simulink model "Controller"  (R2018b)
settings: configuration reference "control_config" (kept outside this file)
values from neighbouring files (symbols this model uses):
  CONTROL_EXPORT = Simulink.Parameter(CONTROL_EXPORT_VALUE)    [controller_model_init.m]
  CONTROL_PARAM = Simulink.Parameter(CONTROL_PARAM_VALUE)    [controller_model_init.m]
undefined symbols (not defined in the file or in its folder): actuator_cmd, ControlMode, DiscIntNeverNeededParam, timestamp
libraries: FMT_Model_Lib x4, simulink x3
settings Model: Creator=jc  LastModifiedBy=zouji
settings ConfigSetRef: SourceLocation=Base Workspace

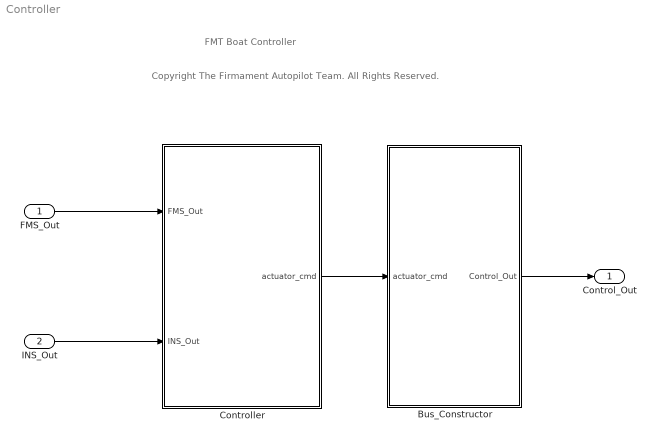
== system Controller ==
  note: FMT Boat Controller
  note: Copyright The Firmament Autopilot Team. All Rights Reserved.
  FMS_Out : Inport  OutDataTypeStr=Bus: FMS_Out_Bus
  INS_Out : Inport  Port=2  OutDataTypeStr=Bus: INS_Out_Bus
  Bus_Constructor : Subsystem
  Controller : Subsystem
  Control_Out : Outport  OutDataTypeStr=Bus: Control_Out_Bus
  wires:
  Bus_Constructor/1(Control_Out) -> Control_Out/1
  INS_Out/1 -> Controller/2(INS_Out)
  FMS_Out/1 -> Controller/1(FMS_Out)
  Controller/1(actuator_cmd) -> Bus_Constructor/1(actuator_cmd)

== system Controller/Bus_Constructor ==
  actuator_cmd : Inport
  Bus Assignment : BusAssignment  AssignedSignals=actuator_cmd,timestamp
  Constant : Constant  Value=0  OutDataTypeStr=Bus: Control_Out_Bus
  timestamp : Subsystem  mask{sample_time=CONTROL_EXPORT.period}
      mask prompts: sample_time "sample time (ms)"
  Control_Out : Outport
  wires:
  actuator_cmd/1 -> Bus Assignment/2
  Constant/1 -> Bus Assignment/1
  Bus Assignment/1 -> Control_Out/1
  timestamp/1(timestamp_ms) -> Bus Assignment/3

== system Controller/Controller ==
  FMS_Out : Inport
  INS_Out : Inport  Port=2
  Control_Allocation : Subsystem  Variant=on
      settings: GeneratePreprocessorConditionals=on
  Heading_Controller : Subsystem
  Speed_Controller : Subsystem
  actuator_cmd : Outport
  wires:
  FMS_Out/1 -> Speed_Controller/1(FMS_Out), Heading_Controller/2(FMS_Out), Control_Allocation/3(FMS_Out)
  INS_Out/1 -> Heading_Controller/1(INS_Out), Speed_Controller/2(INS_Out)
  Control_Allocation/1(actuator_cmd) -> actuator_cmd/1
  Speed_Controller/1(throttle_cmd) -> Control_Allocation/1(throttle_cmd)  "throttle_cmd"
  Heading_Controller/1(steering_cmd) -> Control_Allocation/2(steering_cmd)  "steering_cmd"

== system Controller/Bus_Constructor/timestamp ==
  Constant : Constant  Value=sample_time
  Data Type Conversion : DataTypeConversion  OutDataTypeStr=uint32
  Discrete-Time Integrator : DiscreteIntegrator  IntegratorMethod=Accumulation: Forward Euler  SampleTime=-1  ICPrevOutput=DiscIntNeverNeededParam  ICPrevScaledInput=DiscIntNeverNeededParam
  timestamp_ms : Outport
  wires:
  Discrete-Time Integrator/1 -> Data Type Conversion/1
  Constant/1 -> Discrete-Time Integrator/1
  Data Type Conversion/1 -> timestamp_ms/1

== system Controller/Controller/Control_Allocation ==
  note: 1) Add Subsystem or Model blocks as valid variant choices.
      | 2) You cannot connect blocks at this level. At simulation, connectivity is automatically
      | determined, based on the active variant and port name matching.
  throttle_cmd : Inport
  steering_cmd : Inport  Port=2
  FMS_Out : Inport  Port=3
  Boat_1 : Subsystem  TreatAsAtomicUnit=on  VariantControl=AIRFRAME==1
      mask Display: image('D:\ws\FMT\FMT-Model\figures\boat_1.png');
  Boat_2 : Subsystem  TreatAsAtomicUnit=on  VariantControl=AIRFRAME==2
      mask Display: image('D:\ws\FMT\FMT-Model\figures\boat_1.png');
  actuator_cmd : Outport

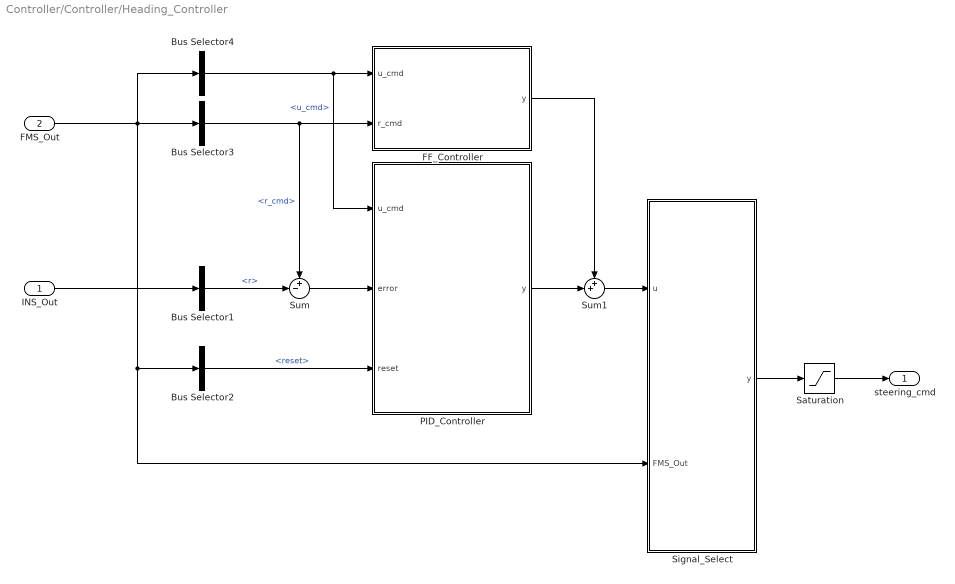
== system Controller/Controller/Heading_Controller ==
  INS_Out : Inport
  FMS_Out : Inport  Port=2
  Bus Selector1 : BusSelector  OutputSignals=r
  Bus Selector2 : BusSelector  OutputSignals=reset
  Bus Selector3 : BusSelector  OutputSignals=r_cmd
  Bus Selector4 : BusSelector  OutputSignals=u_cmd
  FF_Controller : Subsystem
  PID_Controller : Subsystem
  Saturation : Saturate  UpperLimit=1  LowerLimit=-1
  Signal_Select : Subsystem
  Sum : Sum  Inputs=+-|
  Sum1 : Sum  Inputs=++|
  steering_cmd : Outport
  wires:
  Bus Selector2/1 -> PID_Controller/3(reset)  "<reset>"
  Sum/1 -> PID_Controller/2(error)
  FMS_Out/1 -> Bus Selector4/1, Signal_Select/2(FMS_Out), Bus Selector2/1, Bus Selector3/1
  Bus Selector3/1 -> Sum/1, FF_Controller/2(r_cmd)  "<r_cmd>"
  INS_Out/1 -> Bus Selector1/1
  Bus Selector1/1 -> Sum/2  "<r>"
  PID_Controller/1(y) -> Sum1/2
  Signal_Select/1(y) -> Saturation/1
  Saturation/1 -> steering_cmd/1
  Sum1/1 -> Signal_Select/1(u)
  Bus Selector4/1 -> FF_Controller/1(u_cmd), PID_Controller/1(u_cmd)  "<u_cmd>"
  FF_Controller/1(y) -> Sum1/1

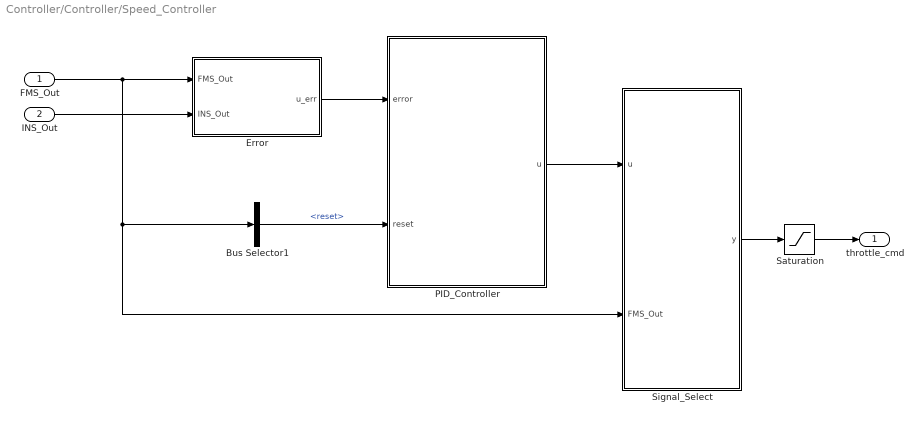
== system Controller/Controller/Speed_Controller ==
  FMS_Out : Inport
  INS_Out : Inport  Port=2
  Bus Selector1 : BusSelector  OutputSignals=reset
  Error : Subsystem
  PID_Controller : Subsystem
  Saturation : Saturate  UpperLimit=1  LowerLimit=-1
  Signal_Select : Subsystem
  throttle_cmd : Outport
  wires:
  Bus Selector1/1 -> PID_Controller/2(reset)  "<reset>"
  FMS_Out/1 -> Signal_Select/2(FMS_Out), Bus Selector1/1, Error/1(FMS_Out)
  Error/1(u_err) -> PID_Controller/1(error)
  PID_Controller/1(u) -> Signal_Select/1(u)
  INS_Out/1 -> Error/2(INS_Out)
  Signal_Select/1(y) -> Saturation/1
  Saturation/1 -> throttle_cmd/1

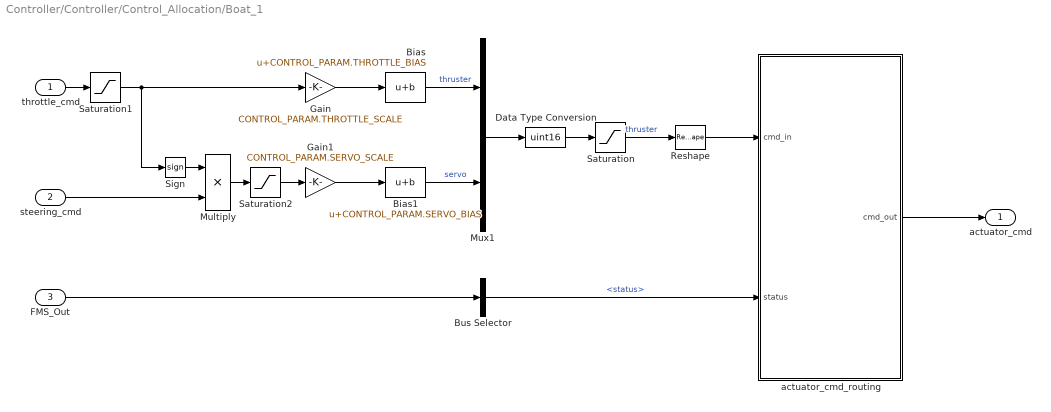
== system Controller/Controller/Control_Allocation/Boat_1 ==
  throttle_cmd : Inport
  steering_cmd : Inport  Port=2
  FMS_Out : Inport  Port=3
  Bias : Bias  Bias=CONTROL_PARAM.THROTTLE_BIAS
  Bias1 : Bias  Bias=CONTROL_PARAM.SERVO_BIAS
  Bus Selector : BusSelector  OutputSignals=status
  Data Type Conversion : DataTypeConversion  OutDataTypeStr=uint16
  Gain : Gain  Gain=CONTROL_PARAM.THROTTLE_SCALE  OutDataTypeStr=single
  Gain1 : Gain  Gain=CONTROL_PARAM.SERVO_SCALE  OutDataTypeStr=single
  Multiply : Product
  Mux1 : Mux  Inputs=2
  Reshape : Reshape  OutputDimensionality=Column vector (2-D)
  Saturation : Saturate  UpperLimit=2000  LowerLimit=1000
  Saturation1 : Saturate  UpperLimit=CONTROL_PARAM.THROTTLE_MAX  LowerLimit=CONTROL_PARAM.THROTTLE_MIN
  Saturation2 : Saturate  UpperLimit=CONTROL_PARAM.SERVO_MAX  LowerLimit=CONTROL_PARAM.SERVO_MIN
  Sign : Signum
  actuator_cmd_routing : Subsystem
  actuator_cmd : Outport
  wires:
  Bias1/1 -> Mux1/2  "servo"
  Gain1/1 -> Bias1/1
  Gain/1 -> Bias/1
  steering_cmd/1 -> Multiply/2
  Bias/1 -> Mux1/1  "thruster"
  Bus Selector/1 -> actuator_cmd_routing/2(status)  "<status>"
  Reshape/1 -> actuator_cmd_routing/1(cmd_in)
  FMS_Out/1 -> Bus Selector/1
  Mux1/1 -> Data Type Conversion/1
  actuator_cmd_routing/1(cmd_out) -> actuator_cmd/1
  Saturation/1 -> Reshape/1  "thruster"
  Data Type Conversion/1 -> Saturation/1
  throttle_cmd/1 -> Saturation1/1
  Saturation2/1 -> Gain1/1
  Multiply/1 -> Saturation2/1
  Sign/1 -> Multiply/1
  Saturation1/1 -> Sign/1, Gain/1

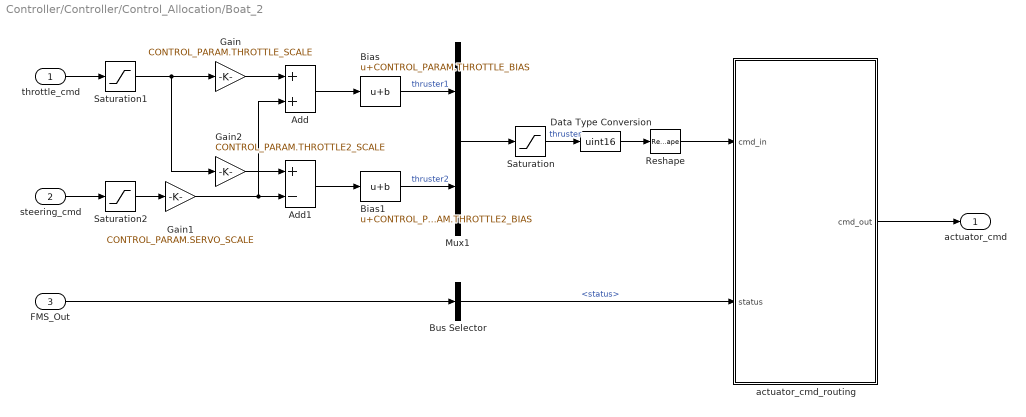
== system Controller/Controller/Control_Allocation/Boat_2 ==
  throttle_cmd : Inport
  steering_cmd : Inport  Port=2
  FMS_Out : Inport  Port=3
  Add : Sum
  Add1 : Sum  Inputs=+-
  Bias : Bias  Bias=CONTROL_PARAM.THROTTLE_BIAS
  Bias1 : Bias  Bias=CONTROL_PARAM.THROTTLE2_BIAS
  Bus Selector : BusSelector  OutputSignals=status
  Data Type Conversion : DataTypeConversion  OutDataTypeStr=uint16
  Gain : Gain  Gain=CONTROL_PARAM.THROTTLE_SCALE  OutDataTypeStr=single
  Gain1 : Gain  Gain=CONTROL_PARAM.SERVO_SCALE  OutDataTypeStr=single
  Gain2 : Gain  Gain=CONTROL_PARAM.THROTTLE2_SCALE  OutDataTypeStr=single
  Mux1 : Mux  Inputs=2
  Reshape : Reshape  OutputDimensionality=Column vector (2-D)
  Saturation : Saturate  UpperLimit=2000  LowerLimit=1000
  Saturation1 : Saturate  UpperLimit=CONTROL_PARAM.THROTTLE_MAX  LowerLimit=CONTROL_PARAM.THROTTLE_MIN
  Saturation2 : Saturate  UpperLimit=CONTROL_PARAM.SERVO_MAX  LowerLimit=CONTROL_PARAM.SERVO_MIN
  actuator_cmd_routing : Subsystem
  actuator_cmd : Outport
  wires:
  Bias1/1 -> Mux1/2  "thruster2"
  throttle_cmd/1 -> Saturation1/1
  Bias/1 -> Mux1/1  "thruster1"
  Bus Selector/1 -> actuator_cmd_routing/2(status)  "<status>"
  Reshape/1 -> actuator_cmd_routing/1(cmd_in)
  FMS_Out/1 -> Bus Selector/1
  actuator_cmd_routing/1(cmd_out) -> actuator_cmd/1
  Saturation/1 -> Data Type Conversion/1  "thruster"
  Mux1/1 -> Saturation/1
  steering_cmd/1 -> Saturation2/1
  Saturation1/1 -> Gain2/1, Gain/1
  Data Type Conversion/1 -> Reshape/1
  Add1/1 -> Bias1/1
  Add/1 -> Bias/1
  Gain/1 -> Add/1
  Gain1/1 -> Add/2, Add1/2
  Saturation2/1 -> Gain1/1
  Gain2/1 -> Add1/1

== system Controller/Controller/Heading_Controller/FF_Controller ==
  u_cmd : Inport
  r_cmd : Inport  Port=2
  BW_FF : Gain  Gain=CONTROL_PARAM.BW_PSI_RATE_FF
  FW_FF : Gain  Gain=CONTROL_PARAM.FW_PSI_RATE_FF
  Saturation : Saturate  UpperLimit=1  LowerLimit=-1
  Switch : Switch
  y : Outport
  wires:
  r_cmd/1 -> BW_FF/1, FW_FF/1
  FW_FF/1 -> Switch/1
  BW_FF/1 -> Switch/3
  Switch/1 -> Saturation/1
  u_cmd/1 -> Switch/2
  Saturation/1 -> y/1

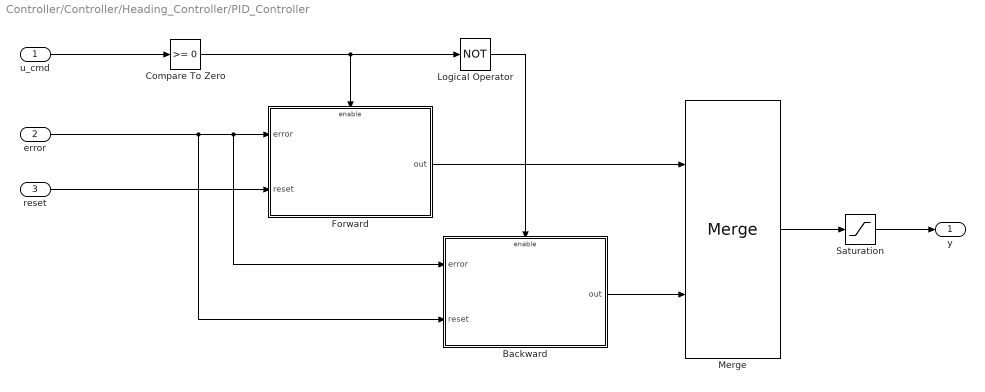
== system Controller/Controller/Heading_Controller/PID_Controller ==
  u_cmd : Inport
  error : Inport  Port=2
  reset : Inport  Port=3
  Backward : Subsystem
  Compare To Zero : simulink/Logic and Bit Operations/Compare To Zero  relop=>=  OutDataTypeStr=boolean
  Forward : Subsystem
  Logical Operator : Logic  Operator=NOT  AllPortsSameDT=off  OutDataTypeStr=boolean
  Merge : Merge
  Saturation : Saturate  UpperLimit=1  LowerLimit=-1
  y : Outport
  wires:
  Saturation/1 -> y/1
  error/1 -> Backward/2(reset), Backward/1(error), Forward/1(error)
  reset/1 -> Forward/2(reset)
  u_cmd/1 -> Compare To Zero/1
  Compare To Zero/1 -> Logical Operator/1, Forward/Enable
  Logical Operator/1 -> Backward/Enable
  Backward/1(out) -> Merge/2
  Forward/1(out) -> Merge/1
  Merge/1 -> Saturation/1

== system Controller/Controller/Heading_Controller/Signal_Select ==
  u : Inport
  FMS_Out : Inport  Port=2
  Bus Selector : BusSelector  OutputSignals=ctrl_mode
  Bus Selector1 : BusSelector  OutputSignals=r_cmd
  Position : simulink/Logic and Bit Operations/Compare To Constant  relop=>=  const=uint8(ControlMode.Stabilize)  OutDataTypeStr=boolean
  Switch : Switch  Criteria=u2 > Threshold
  y : Outport
  wires:
  FMS_Out/1 -> Bus Selector1/1, Bus Selector/1
  Bus Selector/1 -> Position/1  "<ctrl_mode>"
  Position/1 -> Switch/2
  Switch/1 -> y/1
  u/1 -> Switch/1
  Bus Selector1/1 -> Switch/3  "<r_cmd>"

== system Controller/Controller/Speed_Controller/Error ==
  FMS_Out : Inport
  INS_Out : Inport  Port=2
  Bus Selector2 : BusSelector  OutputSignals=u_cmd
  Bus_Select : Subsystem
  Sum : Sum  Inputs=|+-
  u_err : Outport
  wires:
  FMS_Out/1 -> Bus Selector2/1
  INS_Out/1 -> Bus_Select/1(INS_Out)
  Bus_Select/1(u_est_C_mPs) -> Sum/2  "u_est"
  Bus Selector2/1 -> Sum/1  "<u_cmd>"
  Sum/1 -> u_err/1  "u_err"

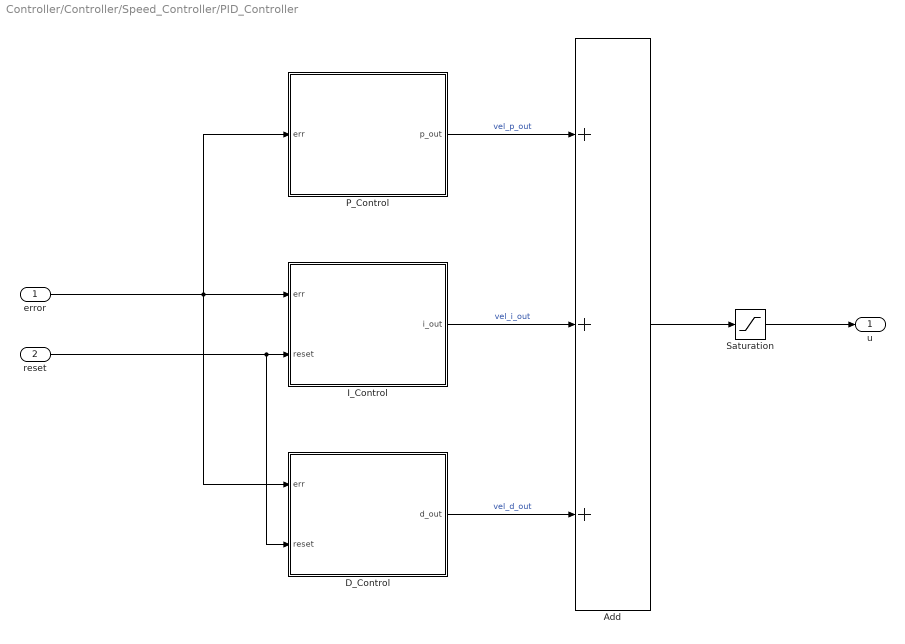
== system Controller/Controller/Speed_Controller/PID_Controller ==
  error : Inport
  reset : Inport  Port=2
  Add : Sum  Inputs=+++
  D_Control : Subsystem  mask{kd=CONTROL_PARAM.VEL_D, max_d=CONTROL_PARAM.VEL_D_MAX, min_d=CONTROL_PARAM.VEL_D_MIN}
  I_Control : Subsystem  mask{ki=CONTROL_PARAM.VEL_I, max_i=CONTROL_PARAM.VEL_I_MAX, min_i=CONTROL_PARAM.VEL_I_MIN}
  P_Control : Subsystem  mask{kp=CONTROL_PARAM.VEL_P}
  Saturation : Saturate  UpperLimit=1  LowerLimit=-1
  u : Outport
  wires:
  error/1 -> P_Control/1(err), I_Control/1(err), D_Control/1(err)
  P_Control/1(p_out) -> Add/1  "vel_p_out"
  I_Control/1(i_out) -> Add/2  "vel_i_out"
  D_Control/1(d_out) -> Add/3  "vel_d_out"
  reset/1 -> I_Control/2(reset), D_Control/2(reset)
  Add/1 -> Saturation/1
  Saturation/1 -> u/1

== system Controller/Controller/Speed_Controller/Signal_Select ==
  u : Inport
  FMS_Out : Inport  Port=2
  Bus Selector : BusSelector  OutputSignals=ctrl_mode
  Bus Selector1 : BusSelector  OutputSignals=u_cmd
  Position : simulink/Logic and Bit Operations/Compare To Constant  relop=>=  const=uint8(ControlMode.POSCTL)  OutDataTypeStr=boolean
  Switch : Switch  Criteria=u2 > Threshold
  y : Outport
  wires:
  FMS_Out/1 -> Bus Selector1/1, Bus Selector/1
  Bus Selector/1 -> Position/1  "<ctrl_mode>"
  Position/1 -> Switch/2
  Switch/1 -> y/1
  u/1 -> Switch/1
  Bus Selector1/1 -> Switch/3  "<u_cmd>"

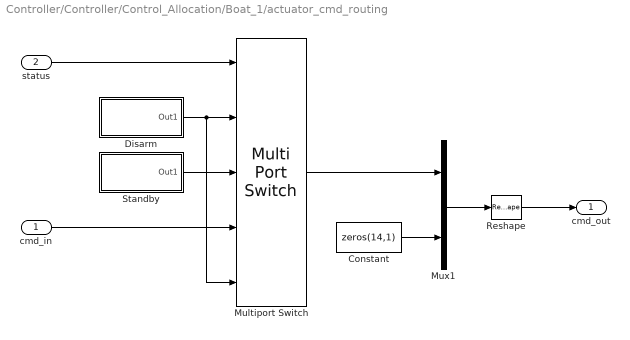
== system Controller/Controller/Control_Allocation/Boat_1/actuator_cmd_routing ==
  cmd_in : Inport
  status : Inport  Port=2
  Constant : Constant  Value=zeros(14,1)  VectorParams1D=off  OutDataTypeStr=uint16
  Disarm : Subsystem
  Multiport Switch : MultiPortSwitch  DataPortForDefault=Additional data port  DiagnosticForDefault=None
  Mux1 : Mux  Inputs=2
  Reshape : Reshape  OutputDimensionality=Customize  OutputDimensions=[16,1]
  Standby : Subsystem
  cmd_out : Outport
  wires:
  Reshape/1 -> cmd_out/1
  Constant/1 -> Mux1/2
  Mux1/1 -> Reshape/1
  status/1 -> Multiport Switch/1
  Multiport Switch/1 -> Mux1/1
  cmd_in/1 -> Multiport Switch/4
  Disarm/1(Out1) -> Multiport Switch/5, Multiport Switch/2
  Standby/1(Out1) -> Multiport Switch/3

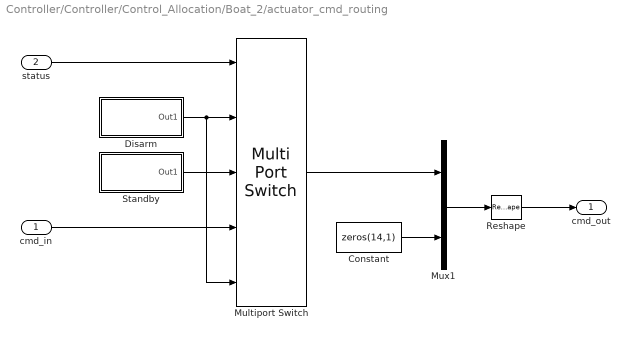
== system Controller/Controller/Control_Allocation/Boat_2/actuator_cmd_routing ==
  cmd_in : Inport
  status : Inport  Port=2
  Constant : Constant  Value=zeros(14,1)  VectorParams1D=off  OutDataTypeStr=uint16
  Disarm : Subsystem
  Multiport Switch : MultiPortSwitch  DataPortForDefault=Additional data port  DiagnosticForDefault=None
  Mux1 : Mux  Inputs=2
  Reshape : Reshape  OutputDimensionality=Customize  OutputDimensions=[16,1]
  Standby : Subsystem
  cmd_out : Outport
  wires:
  Reshape/1 -> cmd_out/1
  Constant/1 -> Mux1/2
  Mux1/1 -> Reshape/1
  status/1 -> Multiport Switch/1
  Multiport Switch/1 -> Mux1/1
  cmd_in/1 -> Multiport Switch/4
  Disarm/1(Out1) -> Multiport Switch/5, Multiport Switch/2
  Standby/1(Out1) -> Multiport Switch/3

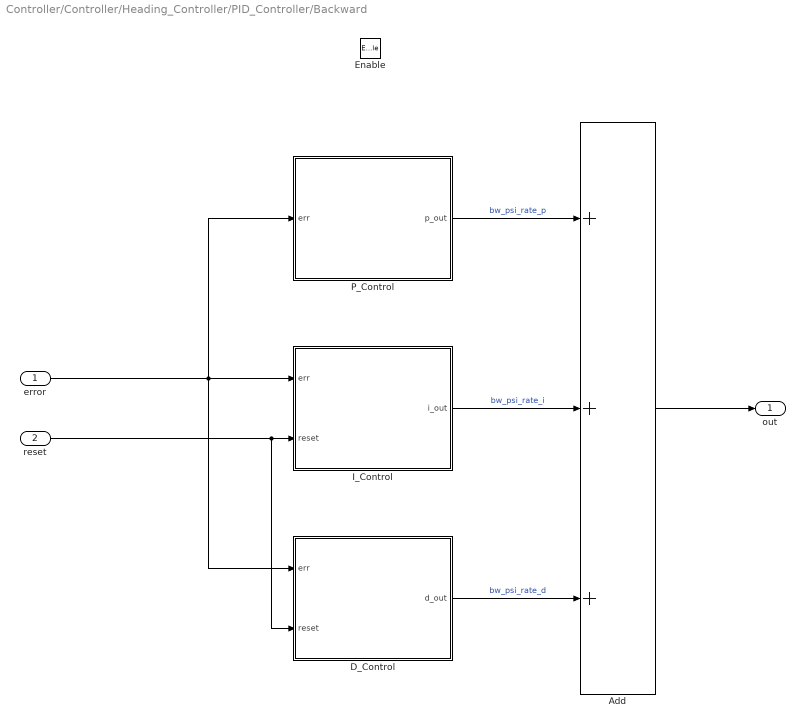
== system Controller/Controller/Heading_Controller/PID_Controller/Backward ==
  error : Inport
  reset : Inport  Port=2
  Enable : EnablePort  StatesWhenEnabling=reset
  Add : Sum  Inputs=+++
  D_Control : Subsystem  mask{kd=CONTROL_PARAM.BW_PSI_RATE_D, max_d=0.2, min_d=-0.2}
  I_Control : Subsystem  mask{ki=CONTROL_PARAM.BW_PSI_RATE_I, max_i=0.2, min_i=-0.2}
  P_Control : Subsystem  mask{kp=CONTROL_PARAM.BW_PSI_RATE_P}
  out : Outport
  wires:
  I_Control/1(i_out) -> Add/2  "bw_psi_rate_i"
  D_Control/1(d_out) -> Add/3  "bw_psi_rate_d"
  Add/1 -> out/1
  reset/1 -> D_Control/2(reset), I_Control/2(reset)
  P_Control/1(p_out) -> Add/1  "bw_psi_rate_p"
  error/1 -> D_Control/1(err), I_Control/1(err), P_Control/1(err)

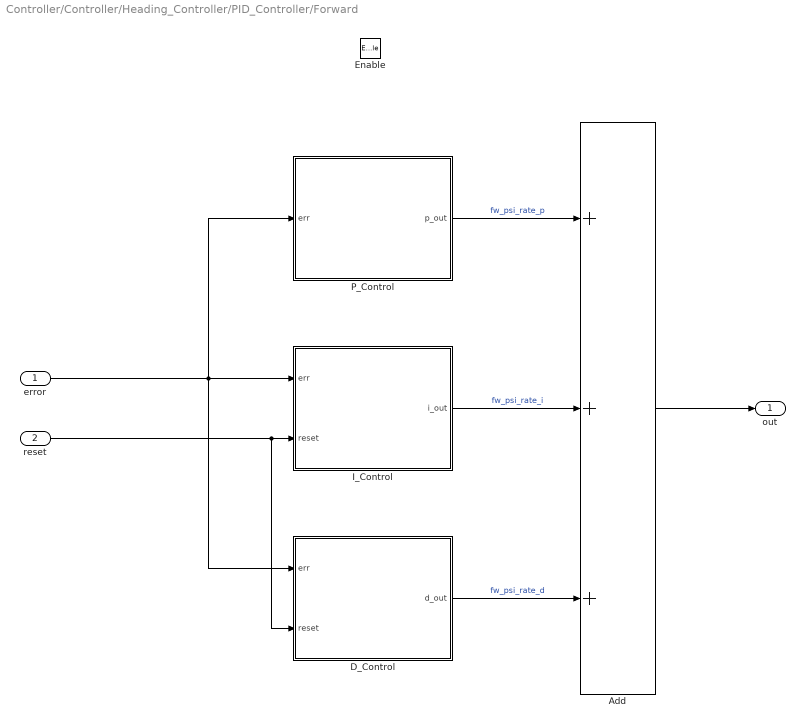
== system Controller/Controller/Heading_Controller/PID_Controller/Forward ==
  error : Inport
  reset : Inport  Port=2
  Enable : EnablePort  StatesWhenEnabling=reset
  Add : Sum  Inputs=+++
  D_Control : Subsystem  mask{kd=CONTROL_PARAM.FW_PSI_RATE_D, max_d=0.2, min_d=-0.2}
  I_Control : Subsystem  mask{ki=CONTROL_PARAM.FW_PSI_RATE_I, max_i=0.2, min_i=-0.2}
  P_Control : Subsystem  mask{kp=CONTROL_PARAM.FW_PSI_RATE_P}
  out : Outport
  wires:
  error/1 -> P_Control/1(err), I_Control/1(err), D_Control/1(err)
  P_Control/1(p_out) -> Add/1  "fw_psi_rate_p"
  reset/1 -> I_Control/2(reset), D_Control/2(reset)
  Add/1 -> out/1
  D_Control/1(d_out) -> Add/3  "fw_psi_rate_d"
  I_Control/1(i_out) -> Add/2  "fw_psi_rate_i"

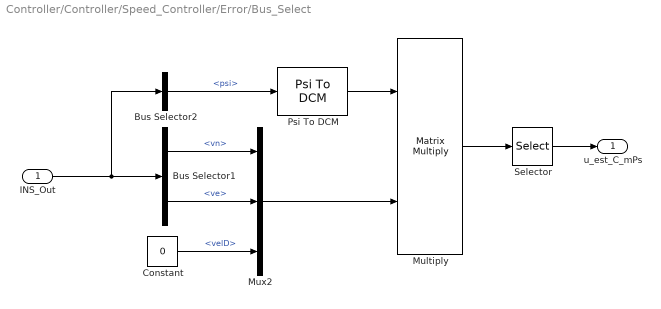
== system Controller/Controller/Speed_Controller/Error/Bus_Select ==
  INS_Out : Inport
  Bus Selector1 : BusSelector  OutputSignals=vn,ve
  Bus Selector2 : BusSelector  OutputSignals=psi
  Constant : Constant  Value=0  OutDataTypeStr=single
  Multiply : Product  Multiplication=Matrix(*)
  Mux2 : Mux  Inputs=3
  Psi To DCM : FMT_Model_Lib/Transformation/Psi To DCM
      settings: SourceProductName=FMT Toolbox
  Selector : Selector  InputPortWidth=3  IndexOptions=Index vector (dialog)  Indices=1  OutputSizes=1
  u_est_C_mPs : Outport
  wires:
  Psi To DCM/1 -> Multiply/1
  Bus Selector2/1 -> Psi To DCM/1  "<psi>"
  Constant/1 -> Mux2/3  "<velD>"
  Mux2/1 -> Multiply/2
  Bus Selector1/2 -> Mux2/2  "<ve>"
  Bus Selector1/1 -> Mux2/1  "<vn>"
  INS_Out/1 -> Bus Selector2/1, Bus Selector1/1
  Multiply/1 -> Selector/1
  Selector/1 -> u_est_C_mPs/1

== system Controller/Controller/Speed_Controller/PID_Controller/D_Control ==
  err : Inport
  reset : Inport  Port=2
  DT Filter : FMT_Model_Lib/Filter/DT Filter  fc=30
      settings: SourceProductName=FMT Toolbox
  Multiply : Product  OutDataTypeStr=Inherit: Same as first input
  Saturation : Saturate  UpperLimit=max_d  LowerLimit=min_d
  gain1 : Constant  Value=kd  OutDataTypeStr=single
  d_out : Outport
  wires:
  err/1 -> DT Filter/1
  Multiply/1 -> Saturation/1
  Saturation/1 -> d_out/1
  reset/1 -> DT Filter/2
  gain1/1 -> Multiply/1
  DT Filter/1 -> Multiply/2

== system Controller/Controller/Speed_Controller/PID_Controller/I_Control ==
  err : Inport
  reset : Inport  Port=2
  Constant : Constant  Value=0  OutDataTypeStr=single
  Discrete-Time Integrator : DiscreteIntegrator  ExternalReset=level  InitialConditionSource=external  SampleTime=-1  LimitOutput=on  UpperSaturationLimit=max_i  LowerSaturationLimit=min_i  ICPrevOutput=DiscIntNeverNeededParam  ICPrevScaledInput=DiscIntNeverNeededParam
  Multiply : Product  OutDataTypeStr=Inherit: Same as first input
  gain1 : Constant  Value=ki  OutDataTypeStr=single
  i_out : Outport
  wires:
  err/1 -> Multiply/2
  reset/1 -> Discrete-Time Integrator/2
  Constant/1 -> Discrete-Time Integrator/3
  Discrete-Time Integrator/1 -> i_out/1
  gain1/1 -> Multiply/1
  Multiply/1 -> Discrete-Time Integrator/1

== system Controller/Controller/Speed_Controller/PID_Controller/P_Control ==
  err : Inport
  Multiply : Product  OutDataTypeStr=Inherit: Same as first input
  gain1 : Constant  Value=kp  OutDataTypeStr=single
  p_out : Outport
  wires:
  err/1 -> Multiply/2
  Multiply/1 -> p_out/1
  gain1/1 -> Multiply/1

== system Controller/Controller/Control_Allocation/Boat_1/actuator_cmd_routing/Disarm ==
  Disarm : Constant  Value=CONTROL_PARAM.THROTTLE_BIAS  VectorParams1D=off  OutDataTypeStr=uint16
  Disarm1 : Constant  Value=CONTROL_PARAM.SERVO_BIAS  VectorParams1D=off  OutDataTypeStr=uint16
  Mux : Mux  Inputs=2
  Out1 : Outport
  wires:
  Mux/1 -> Out1/1
  Disarm/1 -> Mux/1
  Disarm1/1 -> Mux/2

== system Controller/Controller/Control_Allocation/Boat_1/actuator_cmd_routing/Standby ==
  Mux : Mux  Inputs=2
  Standby : Constant  Value=CONTROL_PARAM.THROTTLE_BIAS  VectorParams1D=off  OutDataTypeStr=uint16
  Standby1 : Constant  Value=CONTROL_PARAM.SERVO_BIAS  VectorParams1D=off  OutDataTypeStr=uint16
  Out1 : Outport
  wires:
  Standby/1 -> Mux/1
  Mux/1 -> Out1/1
  Standby1/1 -> Mux/2

== system Controller/Controller/Control_Allocation/Boat_2/actuator_cmd_routing/Disarm ==
  Disarm : Constant  Value=CONTROL_PARAM.THROTTLE_BIAS  VectorParams1D=off  OutDataTypeStr=uint16
  Disarm1 : Constant  Value=CONTROL_PARAM.THROTTLE2_BIAS  VectorParams1D=off  OutDataTypeStr=uint16
  Mux : Mux  Inputs=2
  Out1 : Outport
  wires:
  Mux/1 -> Out1/1
  Disarm/1 -> Mux/1
  Disarm1/1 -> Mux/2

== system Controller/Controller/Control_Allocation/Boat_2/actuator_cmd_routing/Standby ==
  Mux : Mux  Inputs=2
  Standby : Constant  Value=CONTROL_PARAM.THROTTLE_BIAS  VectorParams1D=off  OutDataTypeStr=uint16
  Standby1 : Constant  Value=CONTROL_PARAM.THROTTLE2_BIAS  VectorParams1D=off  OutDataTypeStr=uint16
  Out1 : Outport
  wires:
  Standby/1 -> Mux/1
  Mux/1 -> Out1/1
  Standby1/1 -> Mux/2

== system Controller/Controller/Heading_Controller/PID_Controller/Backward/D_Control ==
  err : Inport
  reset : Inport  Port=2
  DT Filter : FMT_Model_Lib/Filter/DT Filter  fc=30
      settings: SourceProductName=FMT Toolbox
  Multiply : Product  OutDataTypeStr=Inherit: Same as first input
  Saturation : Saturate  UpperLimit=max_d  LowerLimit=min_d
  gain1 : Constant  Value=kd  OutDataTypeStr=single
  d_out : Outport
  wires:
  DT Filter/1 -> Multiply/2
  gain1/1 -> Multiply/1
  reset/1 -> DT Filter/2
  Saturation/1 -> d_out/1
  Multiply/1 -> Saturation/1
  err/1 -> DT Filter/1

== system Controller/Controller/Heading_Controller/PID_Controller/Backward/I_Control ==
  err : Inport
  reset : Inport  Port=2
  Constant : Constant  Value=0  OutDataTypeStr=single
  Discrete-Time Integrator : DiscreteIntegrator  ExternalReset=level  InitialConditionSource=external  SampleTime=-1  LimitOutput=on  UpperSaturationLimit=max_i  LowerSaturationLimit=min_i  ICPrevOutput=DiscIntNeverNeededParam  ICPrevScaledInput=DiscIntNeverNeededParam
  Multiply : Product  OutDataTypeStr=Inherit: Same as first input
  gain1 : Constant  Value=ki  OutDataTypeStr=single
  i_out : Outport
  wires:
  Multiply/1 -> Discrete-Time Integrator/1
  gain1/1 -> Multiply/1
  Discrete-Time Integrator/1 -> i_out/1
  Constant/1 -> Discrete-Time Integrator/3
  reset/1 -> Discrete-Time Integrator/2
  err/1 -> Multiply/2

== system Controller/Controller/Heading_Controller/PID_Controller/Backward/P_Control ==
  err : Inport
  Multiply : Product  OutDataTypeStr=Inherit: Same as first input
  gain1 : Constant  Value=kp  OutDataTypeStr=single
  p_out : Outport
  wires:
  gain1/1 -> Multiply/1
  Multiply/1 -> p_out/1
  err/1 -> Multiply/2

== system Controller/Controller/Heading_Controller/PID_Controller/Forward/D_Control ==
  err : Inport
  reset : Inport  Port=2
  DT Filter : FMT_Model_Lib/Filter/DT Filter  fc=30
      settings: SourceProductName=FMT Toolbox
  Multiply : Product  OutDataTypeStr=Inherit: Same as first input
  Saturation : Saturate  UpperLimit=max_d  LowerLimit=min_d
  gain1 : Constant  Value=kd  OutDataTypeStr=single
  d_out : Outport
  wires:
  err/1 -> DT Filter/1
  Multiply/1 -> Saturation/1
  Saturation/1 -> d_out/1
  reset/1 -> DT Filter/2
  gain1/1 -> Multiply/1
  DT Filter/1 -> Multiply/2

== system Controller/Controller/Heading_Controller/PID_Controller/Forward/I_Control ==
  err : Inport
  reset : Inport  Port=2
  Constant : Constant  Value=0  OutDataTypeStr=single
  Discrete-Time Integrator : DiscreteIntegrator  ExternalReset=level  InitialConditionSource=external  SampleTime=-1  LimitOutput=on  UpperSaturationLimit=max_i  LowerSaturationLimit=min_i  ICPrevOutput=DiscIntNeverNeededParam  ICPrevScaledInput=DiscIntNeverNeededParam
  Multiply : Product  OutDataTypeStr=Inherit: Same as first input
  gain1 : Constant  Value=ki  OutDataTypeStr=single
  i_out : Outport
  wires:
  err/1 -> Multiply/2
  reset/1 -> Discrete-Time Integrator/2
  Constant/1 -> Discrete-Time Integrator/3
  Discrete-Time Integrator/1 -> i_out/1
  gain1/1 -> Multiply/1
  Multiply/1 -> Discrete-Time Integrator/1

== system Controller/Controller/Heading_Controller/PID_Controller/Forward/P_Control ==
  err : Inport
  Multiply : Product  OutDataTypeStr=Inherit: Same as first input
  gain1 : Constant  Value=kp  OutDataTypeStr=single
  p_out : Outport
  wires:
  err/1 -> Multiply/2
  Multiply/1 -> p_out/1
  gain1/1 -> Multiply/1
